simulink model "flightControlSystem"  (R2026b)
settings: Solver=ode3  StopTime=TFinal
PreLoadFcn:
  | InitVars;
  | definePX4ParamsBus;
undefined symbols (not defined in the file): control_power, DiscIntNeverNeededParam, init, MC_PITCHRATE_MAX, MC_ROLLRATE_MAX, MC_YAWRATE_MAX, PX4_Params_Default, SampleTime, timestamp
libraries: px4Utilslib x52, px4uORBlib x10, vrlib x8, aerolibutil x8, simulink x5, sharedutil x3, matrix_library x2, raspberrypiutilitieslib x2, px4Peripheralslib x2, sharedtransform x1, px4Sensorslib x1
(part 3 of 4)

== system flightControlSystem/MultiCopter Controller/Position & Altitude controller/Position controller/thrustToAttitude ==
  note: - Converts thrust vector to desired attitude (roll, pitch, yaw)
      | - Attitude setpoint is calculated so that the thrust vector aligns with desired acceleration
      | - Yaw setpoint (heading) is directly commanded
  thrust_setpoint_NED_3x1 : Inport
  yaw_setpoint_rad : Inport  Port=2
  Abs : Abs  SaturateOnIntegerOverflow=off
  Assignment : Assignment  DiagnosticForDimensions=Warning  IndexOptions=Index vector (dialog)  Indices=[3]  OutputSizes=1  RuntimeRangeChecks=off
  Assignment1 : Assignment  DiagnosticForDimensions=Warning  IndexOptions=Index vector (dialog)  Indices=3  OutputSizes=1  RuntimeRangeChecks=off
  Compare_Norm : RelationalOperator  Operator=<  OutDataTypeStr=boolean  RndMeth=Simplest  InputSameDT=off
  Constant : Constant  Value=eps  SampleTime=-1
  Constant1 : Constant  SampleTime=-1
  Constant2 : Constant  Value=0  SampleTime=-1
  Constant3 : Constant  Value=0.0  SampleTime=-1
  Constant4 : Constant  Value=1e-6  OutDataTypeStr=single  SampleTime=-1
  Constant5 : Constant  Value=single([0;0;1])  OutDataTypeStr=single  SampleTime=-1
  Cos_YawHeading : Trigonometry  Operator=cos
  Cross_BodyX_eq_Y_cross_Z : matrix_library/Cross Product
  Cross_BodyY_eq_Z_cross_Xdes : matrix_library/Cross Product
  Dot_CheckParallel : DotProduct  OutDataTypeStr=Inherit: Inherit via internal rule
  Gain : Gain  Gain=-1
  Gain1 : Gain  Gain=-1
  Mux_HeadingVector_cosYaw_sinYaw_0 : Mux  Inputs=3
  Negate_ThrustBodyFrame : Gain  Gain=-1
  Negate_ThrustForBodyZ : Gain  Gain=-1
  Normalize_BodyY : vrlib/Utilities/Normalize Vector  maxzero=0
  Normalize_BodyZ : vrlib/Utilities/Normalize Vector  maxzero=0
  Relational Operator : RelationalOperator  Operator=<  OutDataTypeStr=boolean  RndMeth=Simplest  InputSameDT=off
  Relational Operator1 : RelationalOperator  Operator=<  OutDataTypeStr=boolean  RndMeth=Simplest  InputSameDT=off
  RotMat_To_Euler_RPY : MATLAB Function  TreatAsAtomicUnit=on
  Selector : Selector  InputPortWidth=3  IndexOptions=Index vector (dialog)  Indices=3  OutputSizes=1  RuntimeRangeChecks=off
  Selector1 : Selector  InputPortWidth=3  IndexOptions=Index vector (dialog)  Indices=3  OutputSizes=1  RuntimeRangeChecks=off
  Sin_YawHeading : Trigonometry
  Switch_Singularity_BodyY : Switch  Criteria=u2 > Threshold  SaturateOnIntegerOverflow=off  InputSameDT=off
  Switch_Singularity_BodyZ : Switch  Criteria=u2 > Threshold  SaturateOnIntegerOverflow=off  InputSameDT=off
  Switch_Singularity_HeadingParallel : Switch  Criteria=u2 > Threshold  SaturateOnIntegerOverflow=off  InputSameDT=off
  ThrustMagnitude_Norm : MATLAB Function  TreatAsAtomicUnit=on
  attitude_euler_rpy_rad : Outport
  thrust_magnitude_normalized : Outport  Port=2
  thrust_body_frame_for_decoupling : Outport  Port=3
  wires:
  Switch_Singularity_HeadingParallel/1 -> Normalize_BodyY/1
  Gain/1 -> Switch_Singularity_BodyY/1
  Gain1/1 -> Assignment1/2
  Negate_ThrustBodyFrame/1 -> Mux_HeadingVector_cosYaw_sinYaw_0/1
  thrust_setpoint_NED_3x1/1 -> Assignment1/1, ThrustMagnitude_Norm/1(u), Negate_ThrustForBodyZ/1
  Constant/1 -> Compare_Norm/2
  Constant1/1 -> Assignment/2
  Selector1/1 -> thrust_body_frame_for_decoupling/1
  Sin_YawHeading/1 -> Negate_ThrustBodyFrame/1
  ThrustMagnitude_Norm/1(y) -> Gain1/1
  Dot_CheckParallel/1 -> Compare_Norm/1
  yaw_setpoint_rad/1 -> Cos_YawHeading/1, Sin_YawHeading/1
  Negate_ThrustForBodyZ/1 -> Dot_CheckParallel/2, Switch_Singularity_BodyZ/3, Assignment/1, Dot_CheckParallel/1
  Assignment/1 -> Switch_Singularity_BodyZ/1
  Assignment1/1 -> Selector1/1, thrust_magnitude_normalized/1
  Cos_YawHeading/1 -> Mux_HeadingVector_cosYaw_sinYaw_0/2
  Compare_Norm/1 -> Switch_Singularity_BodyZ/2
  Constant3/1 -> Relational Operator/2
  Constant2/1 -> Mux_HeadingVector_cosYaw_sinYaw_0/3
  Switch_Singularity_BodyZ/1 -> Normalize_BodyZ/1
  Mux_HeadingVector_cosYaw_sinYaw_0/1 -> Cross_BodyY_eq_Z_cross_Xdes/1
  Normalize_BodyZ/1 -> Cross_BodyX_eq_Y_cross_Z/1, RotMat_To_Euler_RPY/3(body_z), Selector/1, Cross_BodyY_eq_Z_cross_Xdes/2
  Selector/1 -> Abs/1, Relational Operator/1
  Cross_BodyY_eq_Z_cross_Xdes/1 -> Switch_Singularity_BodyY/3, Gain/1
  Abs/1 -> Relational Operator1/1
  Relational Operator1/1 -> Switch_Singularity_HeadingParallel/2
  Constant5/1 -> Switch_Singularity_HeadingParallel/1
  Constant4/1 -> Relational Operator1/2
  Relational Operator/1 -> Switch_Singularity_BodyY/2
  Switch_Singularity_BodyY/1 -> Switch_Singularity_HeadingParallel/3
  Normalize_BodyY/1 -> RotMat_To_Euler_RPY/1(body_x), Cross_BodyX_eq_Y_cross_Z/2
  Cross_BodyX_eq_Y_cross_Z/1 -> RotMat_To_Euler_RPY/2(body_y)
  RotMat_To_Euler_RPY/1(y) -> attitude_euler_rpy_rad/1

== system flightControlSystem/ParamUpdate/HW_ParamUpdate/ReadParams_OnUpdate/AttitudeCtrl_Params ==
  Cast_Mux_MC_ATT_P : DataTypeConversion  OutDataTypeStr=double  SaturateOnIntegerOverflow=off  RndMeth=Floor
  Cast_RP_MC_YAW_WEIGHT : DataTypeConversion  OutDataTypeStr=double  SaturateOnIntegerOverflow=off  RndMeth=Floor
  Mux_MC_ATT_P : Mux  Inputs=3
  RP_MC_ATT_P_1 : px4Utilslib/Read Parameter  ParameterName=MC_ROLL_P  DataType=FLOAT  SampleTime=-1
  RP_MC_ATT_P_2 : px4Utilslib/Read Parameter  ParameterName=MC_PITCH_P  DataType=FLOAT  SampleTime=-1
  RP_MC_ATT_P_3 : px4Utilslib/Read Parameter  ParameterName=MC_YAW_P  DataType=FLOAT  SampleTime=-1
  RP_MC_YAW_WEIGHT : px4Utilslib/Read Parameter  ParameterName=MC_YAW_WEIGHT  DataType=FLOAT  SampleTime=-1
  Term_Status{,1..3} (4 alike) : Terminator
  MC_ATT_P : Outport
  MC_YAW_WEIGHT : Outport  Port=2
  wires:
  RP_MC_ATT_P_3/2 -> Term_Status3/1
  RP_MC_ATT_P_2/2 -> Term_Status2/1
  RP_MC_ATT_P_1/2 -> Term_Status1/1
  RP_MC_YAW_WEIGHT/2 -> Term_Status/1
  RP_MC_ATT_P_3/1 -> Mux_MC_ATT_P/3
  Mux_MC_ATT_P/1 -> Cast_Mux_MC_ATT_P/1
  RP_MC_ATT_P_2/1 -> Mux_MC_ATT_P/2
  Cast_RP_MC_YAW_WEIGHT/1 -> MC_YAW_WEIGHT/1
  RP_MC_YAW_WEIGHT/1 -> Cast_RP_MC_YAW_WEIGHT/1
  Cast_Mux_MC_ATT_P/1 -> MC_ATT_P/1
  RP_MC_ATT_P_1/1 -> Mux_MC_ATT_P/1

== system flightControlSystem/ParamUpdate/HW_ParamUpdate/ReadParams_OnUpdate/Estimator_Params ==
  Cast_RP_MPC_VELD_LP : DataTypeConversion  OutDataTypeStr=double  SaturateOnIntegerOverflow=off  RndMeth=Floor
  EST_NF_BW_Const : Constant  Value=20  SampleTime=-1
  EST_NF_FRQ_Const : Constant  Value=30  SampleTime=-1
  RP_MPC_VELD_LP : px4Utilslib/Read Parameter  ParameterName=MPC_VELD_LP  DataType=FLOAT  SampleTime=-1
  Term_Status : Terminator
  MPC_VELD_LP : Outport
  EST_NF_FRQ : Outport  Port=2
  EST_NF_BW : Outport  Port=3
  wires:
  EST_NF_BW_Const/1 -> EST_NF_BW/1
  RP_MPC_VELD_LP/2 -> Term_Status/1
  Cast_RP_MPC_VELD_LP/1 -> MPC_VELD_LP/1
  RP_MPC_VELD_LP/1 -> Cast_RP_MPC_VELD_LP/1
  EST_NF_FRQ_Const/1 -> EST_NF_FRQ/1

== system flightControlSystem/ParamUpdate/HW_ParamUpdate/ReadParams_OnUpdate/LandingLogic_Params ==
  Cast_RP_MPC_LAND_ALT1 : DataTypeConversion  OutDataTypeStr=double  SaturateOnIntegerOverflow=off  RndMeth=Floor
  Cast_RP_MPC_LAND_ALT2 : DataTypeConversion  OutDataTypeStr=double  SaturateOnIntegerOverflow=off  RndMeth=Floor
  Cast_RP_MPC_LAND_ALT3 : DataTypeConversion  OutDataTypeStr=double  SaturateOnIntegerOverflow=off  RndMeth=Floor
  Cast_RP_MPC_LAND_CRWL : DataTypeConversion  OutDataTypeStr=double  SaturateOnIntegerOverflow=off  RndMeth=Floor
  Cast_RP_MPC_LAND_SPEED : DataTypeConversion  OutDataTypeStr=double  SaturateOnIntegerOverflow=off  RndMeth=Floor
  Cast_RP_MPC_Z_VEL_MAX_DN_LAND : DataTypeConversion  OutDataTypeStr=double  SaturateOnIntegerOverflow=off  RndMeth=Floor
  RP_MPC_LAND_ALT1 : px4Utilslib/Read Parameter  ParameterName=MPC_LAND_ALT1  DataType=FLOAT  SampleTime=-1
  RP_MPC_LAND_ALT2 : px4Utilslib/Read Parameter  ParameterName=MPC_LAND_ALT2  DataType=FLOAT  SampleTime=-1
  RP_MPC_LAND_ALT3 : px4Utilslib/Read Parameter  ParameterName=MPC_LAND_ALT3  DataType=FLOAT  SampleTime=-1
  RP_MPC_LAND_CRWL : px4Utilslib/Read Parameter  ParameterName=MPC_LAND_CRWL  DataType=FLOAT  SampleTime=-1
  RP_MPC_LAND_SPEED : px4Utilslib/Read Parameter  ParameterName=MPC_LAND_SPEED  DataType=FLOAT  SampleTime=-1
  RP_MPC_Z_VEL_MAX_DN_LAND : px4Utilslib/Read Parameter  ParameterName=MPC_Z_VEL_MAX_DN  DataType=FLOAT  SampleTime=-1
  Term_Out{2..3,5..6,8..9} (6 alike) : Terminator
  Term_Status{,1..5} (6 alike) : Terminator
  MPC_LAND_ALT1 : Outport
  MPC_LAND_ALT2 : Outport  Port=2
  MPC_LAND_ALT3 : Outport  Port=3
  MPC_LAND_SPEED : Outport  Port=4
  MPC_LAND_CRWL : Outport  Port=5
  MPC_Z_VEL_MAX_DN_LAND : Outport  Port=6
  wires:
  RP_MPC_Z_VEL_MAX_DN_LAND/2 -> Term_Status5/1
  RP_MPC_LAND_CRWL/2 -> Term_Status4/1
  RP_MPC_LAND_SPEED/2 -> Term_Status3/1
  Cast_RP_MPC_Z_VEL_MAX_DN_LAND/1 -> MPC_Z_VEL_MAX_DN_LAND/1, Term_Out9/1
  Cast_RP_MPC_LAND_CRWL/1 -> MPC_LAND_CRWL/1, Term_Out8/1
  RP_MPC_LAND_ALT3/2 -> Term_Status2/1
  Cast_RP_MPC_LAND_SPEED/1 -> MPC_LAND_SPEED/1, Term_Out6/1
  Cast_RP_MPC_LAND_ALT3/1 -> MPC_LAND_ALT3/1, Term_Out5/1
  RP_MPC_LAND_ALT2/2 -> Term_Status1/1
  Cast_RP_MPC_LAND_ALT2/1 -> MPC_LAND_ALT2/1, Term_Out3/1
  Cast_RP_MPC_LAND_ALT1/1 -> MPC_LAND_ALT1/1, Term_Out2/1
  RP_MPC_LAND_ALT1/2 -> Term_Status/1
  RP_MPC_LAND_CRWL/1 -> Cast_RP_MPC_LAND_CRWL/1
  RP_MPC_LAND_SPEED/1 -> Cast_RP_MPC_LAND_SPEED/1
  RP_MPC_LAND_ALT2/1 -> Cast_RP_MPC_LAND_ALT2/1
  RP_MPC_LAND_ALT3/1 -> Cast_RP_MPC_LAND_ALT3/1
  RP_MPC_Z_VEL_MAX_DN_LAND/1 -> Cast_RP_MPC_Z_VEL_MAX_DN_LAND/1
  RP_MPC_LAND_ALT1/1 -> Cast_RP_MPC_LAND_ALT1/1

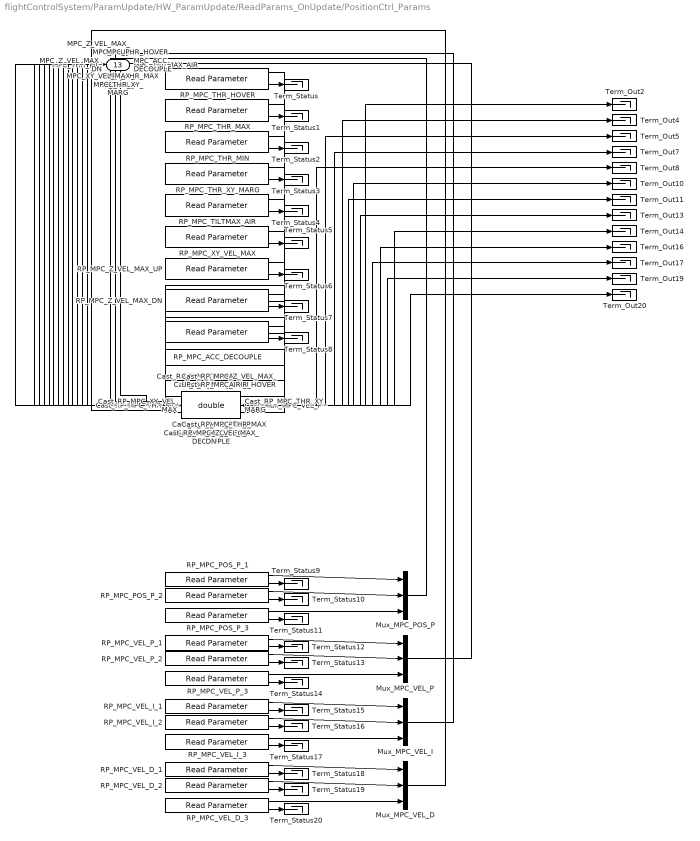
== system flightControlSystem/ParamUpdate/HW_ParamUpdate/ReadParams_OnUpdate/PositionCtrl_Params ==
  Cast_Mux_MPC_POS_P : DataTypeConversion  OutDataTypeStr=double  SaturateOnIntegerOverflow=off  RndMeth=Floor
  Cast_Mux_MPC_VEL_D : DataTypeConversion  OutDataTypeStr=double  SaturateOnIntegerOverflow=off  RndMeth=Floor
  Cast_Mux_MPC_VEL_I : DataTypeConversion  OutDataTypeStr=double  SaturateOnIntegerOverflow=off  RndMeth=Floor
  Cast_Mux_MPC_VEL_P : DataTypeConversion  OutDataTypeStr=double  SaturateOnIntegerOverflow=off  RndMeth=Floor
  Cast_RP_MPC_ACC_DECOUPLE : DataTypeConversion  OutDataTypeStr=double  SaturateOnIntegerOverflow=off  RndMeth=Floor
  Cast_RP_MPC_THR_HOVER : DataTypeConversion  OutDataTypeStr=double  SaturateOnIntegerOverflow=off  RndMeth=Floor
  Cast_RP_MPC_THR_MAX : DataTypeConversion  OutDataTypeStr=double  SaturateOnIntegerOverflow=off  RndMeth=Floor
  Cast_RP_MPC_THR_MIN : DataTypeConversion  OutDataTypeStr=double  SaturateOnIntegerOverflow=off  RndMeth=Floor
  Cast_RP_MPC_THR_XY_MARG : DataTypeConversion  OutDataTypeStr=double  SaturateOnIntegerOverflow=off  RndMeth=Floor
  Cast_RP_MPC_TILTMAX_AIR : DataTypeConversion  OutDataTypeStr=double  SaturateOnIntegerOverflow=off  RndMeth=Floor
  Cast_RP_MPC_XY_VEL_MAX : DataTypeConversion  OutDataTypeStr=double  SaturateOnIntegerOverflow=off  RndMeth=Floor
  Cast_RP_MPC_Z_VEL_MAX_DN : DataTypeConversion  OutDataTypeStr=double  SaturateOnIntegerOverflow=off  RndMeth=Floor
  Cast_RP_MPC_Z_VEL_MAX_UP : DataTypeConversion  OutDataTypeStr=double  SaturateOnIntegerOverflow=off  RndMeth=Floor
  Mux_MPC_POS_P : Mux  Inputs=3
  Mux_MPC_VEL_D : Mux  Inputs=3
  Mux_MPC_VEL_I : Mux  Inputs=3
  Mux_MPC_VEL_P : Mux  Inputs=3
  RP_MPC_ACC_DECOUPLE : px4Utilslib/Read Parameter  ParameterName=MPC_ACC_DECOUPLE  DataType=INT32  SampleTime=-1
  RP_MPC_POS_P_1 : px4Utilslib/Read Parameter  ParameterName=MPC_XY_P  DataType=FLOAT  SampleTime=-1
  RP_MPC_POS_P_2 : px4Utilslib/Read Parameter  ParameterName=MPC_XY_P  DataType=FLOAT  SampleTime=-1
  RP_MPC_POS_P_3 : px4Utilslib/Read Parameter  ParameterName=MPC_Z_P  DataType=FLOAT  SampleTime=-1
  RP_MPC_THR_HOVER : px4Utilslib/Read Parameter  ParameterName=MPC_THR_HOVER  DataType=FLOAT  SampleTime=-1
  RP_MPC_THR_MAX : px4Utilslib/Read Parameter  ParameterName=MPC_THR_MAX  DataType=FLOAT  SampleTime=-1
  RP_MPC_THR_MIN : px4Utilslib/Read Parameter  ParameterName=MPC_THR_MIN  DataType=FLOAT  SampleTime=-1
  RP_MPC_THR_XY_MARG : px4Utilslib/Read Parameter  ParameterName=MPC_THR_XY_MARG  DataType=FLOAT  SampleTime=-1
  RP_MPC_TILTMAX_AIR : px4Utilslib/Read Parameter  ParameterName=MPC_TILTMAX_AIR  DataType=FLOAT  SampleTime=-1
  RP_MPC_VEL_D_1 : px4Utilslib/Read Parameter  ParameterName=MPC_XY_VEL_D_ACC  DataType=FLOAT  SampleTime=-1
  RP_MPC_VEL_D_2 : px4Utilslib/Read Parameter  ParameterName=MPC_XY_VEL_D_ACC  DataType=FLOAT  SampleTime=-1
  RP_MPC_VEL_D_3 : px4Utilslib/Read Parameter  ParameterName=MPC_Z_VEL_D_ACC  DataType=FLOAT  SampleTime=-1
  RP_MPC_VEL_I_1 : px4Utilslib/Read Parameter  ParameterName=MPC_XY_VEL_I_ACC  DataType=FLOAT  SampleTime=-1
  RP_MPC_VEL_I_2 : px4Utilslib/Read Parameter  ParameterName=MPC_XY_VEL_I_ACC  DataType=FLOAT  SampleTime=-1
  RP_MPC_VEL_I_3 : px4Utilslib/Read Parameter  ParameterName=MPC_Z_VEL_I_ACC  DataType=FLOAT  SampleTime=-1
  RP_MPC_VEL_P_1 : px4Utilslib/Read Parameter  ParameterName=MPC_XY_VEL_P_ACC  DataType=FLOAT  SampleTime=-1
  RP_MPC_VEL_P_2 : px4Utilslib/Read Parameter  ParameterName=MPC_XY_VEL_P_ACC  DataType=FLOAT  SampleTime=-1
  RP_MPC_VEL_P_3 : px4Utilslib/Read Parameter  ParameterName=MPC_Z_VEL_P_ACC  DataType=FLOAT  SampleTime=-1
  RP_MPC_XY_VEL_MAX : px4Utilslib/Read Parameter  ParameterName=MPC_XY_VEL_MAX  DataType=FLOAT  SampleTime=-1
  RP_MPC_Z_VEL_MAX_DN : px4Utilslib/Read Parameter  ParameterName=MPC_Z_VEL_MAX_DN  DataType=FLOAT  SampleTime=-1
  RP_MPC_Z_VEL_MAX_UP : px4Utilslib/Read Parameter  ParameterName=MPC_Z_VEL_MAX_UP  DataType=FLOAT  SampleTime=-1
  Term_Out{2,4..5,7..8,10..11,13..14,16..17,19..20} (13 alike) : Terminator
  Term_Status{,1..20} (21 alike) : Terminator
  MPC_POS_P : Outport
  MPC_VEL_P : Outport  Port=2
  MPC_VEL_I : Outport  Port=3
  MPC_VEL_D : Outport  Port=4
  MPC_THR_HOVER : Outport  Port=5
  MPC_THR_MAX : Outport  Port=6
  MPC_THR_MIN : Outport  Port=7
  MPC_THR_XY_MARG : Outport  Port=8
  MPC_TILTMAX_AIR : Outport  Port=9
  MPC_XY_VEL_MAX : Outport  Port=10
  MPC_Z_VEL_MAX_UP : Outport  Port=11
  MPC_Z_VEL_MAX_DN : Outport  Port=12
  MPC_ACC_DECOUPLE : Outport  Port=13
  wires:
  RP_MPC_VEL_D_3/2 -> Term_Status20/1
  RP_MPC_VEL_D_2/2 -> Term_Status19/1
  RP_MPC_VEL_D_1/2 -> Term_Status18/1
  RP_MPC_VEL_I_3/2 -> Term_Status17/1
  RP_MPC_VEL_I_2/2 -> Term_Status16/1
  RP_MPC_VEL_I_1/2 -> Term_Status15/1
  RP_MPC_VEL_P_3/2 -> Term_Status14/1
  RP_MPC_VEL_P_2/2 -> Term_Status13/1
  RP_MPC_VEL_P_1/2 -> Term_Status12/1
  RP_MPC_POS_P_3/2 -> Term_Status11/1
  RP_MPC_POS_P_2/2 -> Term_Status10/1
  RP_MPC_POS_P_1/2 -> Term_Status9/1
  RP_MPC_ACC_DECOUPLE/2 -> Term_Status8/1
  RP_MPC_Z_VEL_MAX_DN/2 -> Term_Status7/1
  Cast_RP_MPC_ACC_DECOUPLE/1 -> MPC_ACC_DECOUPLE/1, Term_Out20/1
  Cast_RP_MPC_Z_VEL_MAX_DN/1 -> MPC_Z_VEL_MAX_DN/1, Term_Out19/1
  RP_MPC_Z_VEL_MAX_UP/2 -> Term_Status6/1
  Cast_RP_MPC_Z_VEL_MAX_UP/1 -> MPC_Z_VEL_MAX_UP/1, Term_Out17/1
  Cast_RP_MPC_XY_VEL_MAX/1 -> MPC_XY_VEL_MAX/1, Term_Out16/1
  RP_MPC_XY_VEL_MAX/2 -> Term_Status5/1
  Cast_RP_MPC_TILTMAX_AIR/1 -> MPC_TILTMAX_AIR/1, Term_Out14/1
  Cast_RP_MPC_THR_XY_MARG/1 -> MPC_THR_XY_MARG/1, Term_Out13/1
  RP_MPC_TILTMAX_AIR/2 -> Term_Status4/1
  Cast_RP_MPC_THR_MIN/1 -> MPC_THR_MIN/1, Term_Out11/1
  Cast_RP_MPC_THR_MAX/1 -> MPC_THR_MAX/1, Term_Out10/1
  RP_MPC_THR_XY_MARG/2 -> Term_Status3/1
  Cast_RP_MPC_THR_HOVER/1 -> MPC_THR_HOVER/1, Term_Out8/1
  Cast_Mux_MPC_VEL_D/1 -> MPC_VEL_D/1, Term_Out7/1
  RP_MPC_THR_MIN/2 -> Term_Status2/1
  Cast_Mux_MPC_VEL_I/1 -> MPC_VEL_I/1, Term_Out5/1
  Cast_Mux_MPC_VEL_P/1 -> MPC_VEL_P/1, Term_Out4/1
  RP_MPC_THR_MAX/2 -> Term_Status1/1
  Cast_Mux_MPC_POS_P/1 -> MPC_POS_P/1, Term_Out2/1
  RP_MPC_THR_HOVER/2 -> Term_Status/1
  RP_MPC_VEL_D_2/1 -> Mux_MPC_VEL_D/2
  RP_MPC_VEL_P_3/1 -> Mux_MPC_VEL_P/3
  RP_MPC_VEL_I_2/1 -> Mux_MPC_VEL_I/2
  Mux_MPC_VEL_P/1 -> Cast_Mux_MPC_VEL_P/1
  Mux_MPC_POS_P/1 -> Cast_Mux_MPC_POS_P/1
  RP_MPC_POS_P_2/1 -> Mux_MPC_POS_P/2
  Mux_MPC_VEL_I/1 -> Cast_Mux_MPC_VEL_I/1
  RP_MPC_POS_P_1/1 -> Mux_MPC_POS_P/1
  RP_MPC_VEL_I_1/1 -> Mux_MPC_VEL_I/1
  RP_MPC_Z_VEL_MAX_DN/1 -> Cast_RP_MPC_Z_VEL_MAX_DN/1
  RP_MPC_THR_XY_MARG/1 -> Cast_RP_MPC_THR_XY_MARG/1
  RP_MPC_POS_P_3/1 -> Mux_MPC_POS_P/3
  Mux_MPC_VEL_D/1 -> Cast_Mux_MPC_VEL_D/1
  RP_MPC_VEL_D_1/1 -> Mux_MPC_VEL_D/1
  RP_MPC_THR_MIN/1 -> Cast_RP_MPC_THR_MIN/1
  RP_MPC_THR_MAX/1 -> Cast_RP_MPC_THR_MAX/1
  RP_MPC_Z_VEL_MAX_UP/1 -> Cast_RP_MPC_Z_VEL_MAX_UP/1
  RP_MPC_VEL_I_3/1 -> Mux_MPC_VEL_I/3
  RP_MPC_VEL_D_3/1 -> Mux_MPC_VEL_D/3
  RP_MPC_VEL_P_1/1 -> Mux_MPC_VEL_P/1
  RP_MPC_ACC_DECOUPLE/1 -> Cast_RP_MPC_ACC_DECOUPLE/1
  RP_MPC_THR_HOVER/1 -> Cast_RP_MPC_THR_HOVER/1
  RP_MPC_XY_VEL_MAX/1 -> Cast_RP_MPC_XY_VEL_MAX/1
  RP_MPC_VEL_P_2/1 -> Mux_MPC_VEL_P/2
  RP_MPC_TILTMAX_AIR/1 -> Cast_RP_MPC_TILTMAX_AIR/1

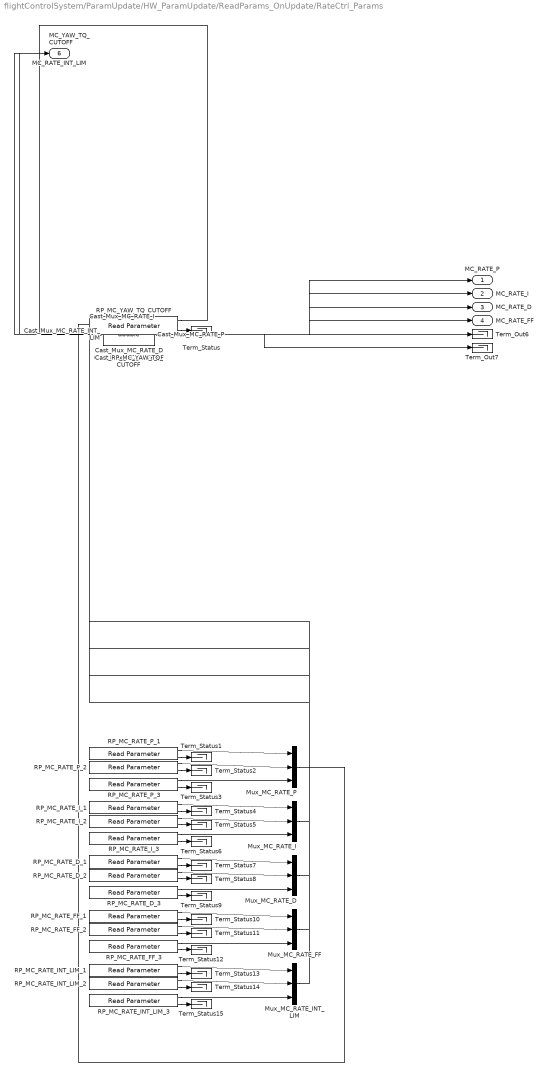
== system flightControlSystem/ParamUpdate/HW_ParamUpdate/ReadParams_OnUpdate/RateCtrl_Params ==
  Cast_Mux_MC_RATE_D : DataTypeConversion  OutDataTypeStr=double  SaturateOnIntegerOverflow=off  RndMeth=Floor
  Cast_Mux_MC_RATE_FF : DataTypeConversion  OutDataTypeStr=double  SaturateOnIntegerOverflow=off  RndMeth=Floor
  Cast_Mux_MC_RATE_I : DataTypeConversion  OutDataTypeStr=double  SaturateOnIntegerOverflow=off  RndMeth=Floor
  Cast_Mux_MC_RATE_INT_LIM : DataTypeConversion  OutDataTypeStr=double  SaturateOnIntegerOverflow=off  RndMeth=Floor
  Cast_Mux_MC_RATE_P : DataTypeConversion  OutDataTypeStr=double  SaturateOnIntegerOverflow=off  RndMeth=Floor
  Cast_RP_MC_YAW_TQ_CUTOFF : DataTypeConversion  OutDataTypeStr=double  SaturateOnIntegerOverflow=off  RndMeth=Floor
  Mux_MC_RATE_D : Mux  Inputs=3
  Mux_MC_RATE_FF : Mux  Inputs=3
  Mux_MC_RATE_I : Mux  Inputs=3
  Mux_MC_RATE_INT_LIM : Mux  Inputs=3
  Mux_MC_RATE_P : Mux  Inputs=3
  RP_MC_RATE_D_1 : px4Utilslib/Read Parameter  ParameterName=MC_ROLLRATE_D  DataType=FLOAT  SampleTime=-1
  RP_MC_RATE_D_2 : px4Utilslib/Read Parameter  ParameterName=MC_PITCHRATE_D  DataType=FLOAT  SampleTime=-1
  RP_MC_RATE_D_3 : px4Utilslib/Read Parameter  ParameterName=MC_YAWRATE_D  DataType=FLOAT  SampleTime=-1
  RP_MC_RATE_FF_1 : px4Utilslib/Read Parameter  ParameterName=MC_ROLLRATE_FF  DataType=FLOAT  SampleTime=-1
  RP_MC_RATE_FF_2 : px4Utilslib/Read Parameter  ParameterName=MC_PITCHRATE_FF  DataType=FLOAT  SampleTime=-1
  RP_MC_RATE_FF_3 : px4Utilslib/Read Parameter  ParameterName=MC_YAWRATE_FF  DataType=FLOAT  SampleTime=-1
  RP_MC_RATE_INT_LIM_1 : px4Utilslib/Read Parameter  ParameterName=MC_RR_INT_LIM  DataType=FLOAT  SampleTime=-1
  RP_MC_RATE_INT_LIM_2 : px4Utilslib/Read Parameter  ParameterName=MC_PR_INT_LIM  DataType=FLOAT  SampleTime=-1
  RP_MC_RATE_INT_LIM_3 : px4Utilslib/Read Parameter  ParameterName=MC_YR_INT_LIM  DataType=FLOAT  SampleTime=-1
  RP_MC_RATE_I_1 : px4Utilslib/Read Parameter  ParameterName=MC_ROLLRATE_I  DataType=FLOAT  SampleTime=-1
  RP_MC_RATE_I_2 : px4Utilslib/Read Parameter  ParameterName=MC_PITCHRATE_I  DataType=FLOAT  SampleTime=-1
  RP_MC_RATE_I_3 : px4Utilslib/Read Parameter  ParameterName=MC_YAWRATE_I  DataType=FLOAT  SampleTime=-1
  RP_MC_RATE_P_1 : px4Utilslib/Read Parameter  ParameterName=MC_ROLLRATE_P  DataType=FLOAT  SampleTime=-1
  RP_MC_RATE_P_2 : px4Utilslib/Read Parameter  ParameterName=MC_PITCHRATE_P  DataType=FLOAT  SampleTime=-1
  RP_MC_RATE_P_3 : px4Utilslib/Read Parameter  ParameterName=MC_YAWRATE_P  DataType=FLOAT  SampleTime=-1
  RP_MC_YAW_TQ_CUTOFF : px4Utilslib/Read Parameter  ParameterName=MC_YAW_TQ_CUTOFF  DataType=FLOAT  SampleTime=-1
  Term_Out6 : Terminator
  Term_Out7 : Terminator
  Term_Status{,1..15} (16 alike) : Terminator
  MC_RATE_P : Outport
  MC_RATE_I : Outport  Port=2
  MC_RATE_D : Outport  Port=3
  MC_RATE_FF : Outport  Port=4
  MC_RATE_INT_LIM : Outport  Port=5
  MC_YAW_TQ_CUTOFF : Outport  Port=6
  wires:
  RP_MC_RATE_INT_LIM_3/2 -> Term_Status15/1
  RP_MC_RATE_INT_LIM_2/2 -> Term_Status14/1
  RP_MC_RATE_INT_LIM_1/2 -> Term_Status13/1
  RP_MC_RATE_FF_3/2 -> Term_Status12/1
  RP_MC_RATE_FF_2/2 -> Term_Status11/1
  RP_MC_RATE_FF_1/2 -> Term_Status10/1
  RP_MC_RATE_D_3/2 -> Term_Status9/1
  RP_MC_RATE_D_2/2 -> Term_Status8/1
  RP_MC_RATE_D_1/2 -> Term_Status7/1
  RP_MC_RATE_I_3/2 -> Term_Status6/1
  RP_MC_RATE_I_2/2 -> Term_Status5/1
  RP_MC_RATE_I_1/2 -> Term_Status4/1
  RP_MC_RATE_P_3/2 -> Term_Status3/1
  RP_MC_RATE_P_2/2 -> Term_Status2/1
  RP_MC_RATE_P_1/2 -> Term_Status1/1
  Cast_RP_MC_YAW_TQ_CUTOFF/1 -> MC_YAW_TQ_CUTOFF/1, Term_Out7/1
  Cast_Mux_MC_RATE_INT_LIM/1 -> MC_RATE_INT_LIM/1, Term_Out6/1
  RP_MC_YAW_TQ_CUTOFF/2 -> Term_Status/1
  Cast_Mux_MC_RATE_D/1 -> MC_RATE_D/1
  Cast_Mux_MC_RATE_I/1 -> MC_RATE_I/1
  Cast_Mux_MC_RATE_P/1 -> MC_RATE_P/1
  Mux_MC_RATE_INT_LIM/1 -> Cast_Mux_MC_RATE_INT_LIM/1
  RP_MC_RATE_INT_LIM_1/1 -> Mux_MC_RATE_INT_LIM/1
  RP_MC_RATE_FF_3/1 -> Mux_MC_RATE_FF/3
  Mux_MC_RATE_FF/1 -> Cast_Mux_MC_RATE_FF/1
  RP_MC_RATE_FF_2/1 -> Mux_MC_RATE_FF/2
  RP_MC_RATE_INT_LIM_2/1 -> Mux_MC_RATE_INT_LIM/2
  RP_MC_RATE_I_3/1 -> Mux_MC_RATE_I/3
  Mux_MC_RATE_I/1 -> Cast_Mux_MC_RATE_I/1
  RP_MC_RATE_I_1/1 -> Mux_MC_RATE_I/1
  RP_MC_RATE_D_2/1 -> Mux_MC_RATE_D/2
  Mux_MC_RATE_D/1 -> Cast_Mux_MC_RATE_D/1
  RP_MC_RATE_INT_LIM_3/1 -> Mux_MC_RATE_INT_LIM/3
  RP_MC_RATE_P_3/1 -> Mux_MC_RATE_P/3
  RP_MC_RATE_I_2/1 -> Mux_MC_RATE_I/2
  RP_MC_RATE_D_3/1 -> Mux_MC_RATE_D/3
  Mux_MC_RATE_P/1 -> Cast_Mux_MC_RATE_P/1
  RP_MC_RATE_P_2/1 -> Mux_MC_RATE_P/2
  RP_MC_RATE_D_1/1 -> Mux_MC_RATE_D/1
  RP_MC_YAW_TQ_CUTOFF/1 -> Cast_RP_MC_YAW_TQ_CUTOFF/1
  Cast_Mux_MC_RATE_FF/1 -> MC_RATE_FF/1
  RP_MC_RATE_P_1/1 -> Mux_MC_RATE_P/1
  RP_MC_RATE_FF_1/1 -> Mux_MC_RATE_FF/1

== system flightControlSystem/SetpointManager/Set target Position/Setpoints from Perception Module/Enabled Subsystem ==
  CurrentPosition : Inport
  Enable : EnablePort
  Cast To Single : DataTypeConversion  OutDataTypeStr=single  SaturateOnIntegerOverflow=off  RndMeth=Floor
  Constant : Constant  Value=221  OutDataTypeStr=single  SampleTime=-1
  Demux : Demux
  Protocol Encoder : raspberrypiutilitieslib/Protocol Encoder  Header=[123]  FieldTable={ 'Field1', '1', 'single', 'Little endian'; 'Field2', '1', 'single', 'Little endian'; 'Field3', '1', 'single', 'Little endian'; 'Field4', '1', 'single', 'Little endian'; 'Field5', '1', 'single', 'Little endian' }  IsChecksumRequired=off  ChecksumAlgorithm=XOR of bytes  ChecksumSize=[]  TerminatorOption=<none>  CustomTerminatorVal=[]
  Selector : Selector  InputPortWidth=5  IndexOptions=Index vector (dialog)  Indices=[1:4]  OutputSizes=1  RuntimeRangeChecks=off
  Serial Transmit : px4Peripheralslib/Serial Transmit  SCIModule=/dev/ttyACM0
  wires:
  CurrentPosition/1 -> Selector/1
  Cast To Single/1 -> Demux/1
  Constant/1 -> Protocol Encoder/5
  Selector/1 -> Cast To Single/1
  Demux/1 -> Protocol Encoder/1
  Demux/2 -> Protocol Encoder/2
  Demux/3 -> Protocol Encoder/3
  Demux/4 -> Protocol Encoder/4
  Protocol Encoder/1 -> Serial Transmit/1

== system flightControlSystem/MultiCopter Controller/Angular Rate Control/RatePID_Core/ActuatorSaturation_Detector/If Action Subsystem1 ==
  Action Port : ActionPort  ActionPortLabel=else
  Constant1 : Constant  Value=[0, 0, 0]  OutDataTypeStr=boolean  SampleTime=-1
  Constant2 : Constant  Value=[0, 0, 0]  OutDataTypeStr=boolean  SampleTime=-1
  saturation_positive : Outport
  saturation_negative : Outport  Port=2
  wires:
  Constant2/1 -> saturation_positive/1
  Constant1/1 -> saturation_negative/1

== system flightControlSystem/MultiCopter Controller/Angular Rate Control/RatePID_Core/ActuatorSaturation_Detector/Subsystem1 ==
  unallocated_torque : Inport
  Action Port : ActionPort  ActionPortLabel=if(u1 ~= 0)
  Constant1 : Constant  Value=eps  SampleTime=-1
  Constant3 : Constant  Value=-eps  SampleTime=-1
  Relational Operator1 : RelationalOperator  Operator=>  OutDataTypeStr=boolean  RndMeth=Simplest  InputSameDT=off
  Relational Operator2 : RelationalOperator  Operator=<  OutDataTypeStr=boolean  RndMeth=Simplest  InputSameDT=off
  saturation_positive : Outport
  saturation_negative : Outport  Port=2
  wires:
  Relational Operator2/1 -> saturation_negative/1
  Constant1/1 -> Relational Operator1/2
  unallocated_torque/1 -> Relational Operator2/1, Relational Operator1/1
  Constant3/1 -> Relational Operator2/2
  Relational Operator1/1 -> saturation_positive/1

== system flightControlSystem/MultiCopter Controller/Angular Rate Control/RatePID_Core/rate_integral/AntiWindup_IntegralUpdate ==
  is_saturated_positive_3x1 : Inport
  is_saturated_negative_3x1 : Inport  Port=2
  gain_I_per_axis : Inport  Port=3
  integral_limit_symmetric : Inport  Port=4
  rate_error_rads : Inport  Port=5
  integral_state_prev : Inport  Port=6
  dt_s : Inport  Port=7
  Action Port : ActionPort  ActionPortLabel=if(u1 ~=0)
  Update_Integral : Subsystem  TreatAsAtomicUnit=on
  integral_state_new : Outport
  wires:
  rate_error_rads/1 -> Update_Integral/5(rate_error_scalar_rads)
  is_saturated_positive_3x1/1 -> Update_Integral/1(saturated_positive_bool)
  integral_state_prev/1 -> Update_Integral/6(integral_prev_scalar)
  is_saturated_negative_3x1/1 -> Update_Integral/2(saturated_negative_bool)
  gain_I_per_axis/1 -> Update_Integral/3(I_gain_scalar)
  dt_s/1 -> Update_Integral/7(dt_s)
  integral_limit_symmetric/1 -> Update_Integral/4(integral_limit)
  Update_Integral/1(integral_updated_scalar) -> integral_state_new/1

== system flightControlSystem/MultiCopter Controller/Angular Rate Control/RatePID_Core/rate_integral/IfLanded_ResetIntegral_PassZero ==
  rate_int_in : Inport
  Action Port : ActionPort  ActionPortLabel=else
  Out1 : Outport
  wires:
  rate_int_in/1 -> Out1/1

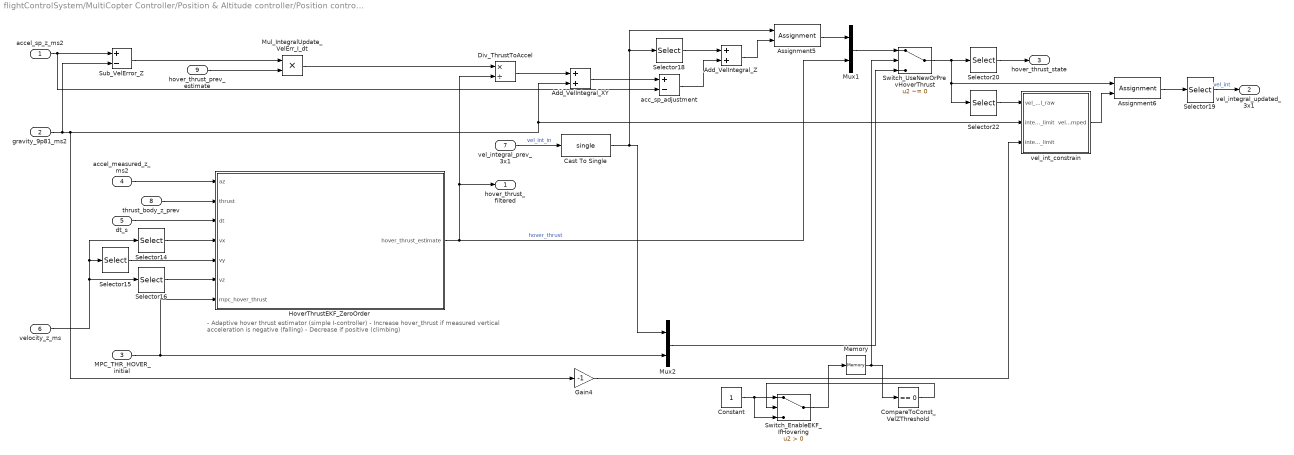
== system flightControlSystem/MultiCopter Controller/Position & Altitude controller/Position controller/PositionVelocityControl/Hover_Thrust ==
  note: - Adaptive hover thrust estimator (simple I-controller)
      | - Increase hover_thrust if measured vertical acceleration is negative (falling)
      | - Decrease if positive (climbing)
  accel_sp_z_ms2 : Inport
  gravity_9p81_ms2 : Inport  Port=2
  MPC_THR_HOVER_initial : Inport  Port=3
  accel_measured_z_ms2 : Inport  Port=4
  dt_s : Inport  Port=5
  velocity_z_ms : Inport  Port=6
  vel_integral_prev_3x1 : Inport  Port=7
  thrust_body_z_prev : Inport  Port=8
  hover_thrust_prev_estimate : Inport  Port=9
  Add_VelIntegral_XY : Sum
  Add_VelIntegral_Z : Sum
  Assignment5 : Assignment  DiagnosticForDimensions=Warning  IndexOptions=Index vector (dialog)  Indices=3  OutputSizes=1  RuntimeRangeChecks=off
  Assignment6 : Assignment  DiagnosticForDimensions=Warning  IndexOptions=Index vector (dialog)  Indices=3  OutputSizes=1  RuntimeRangeChecks=off
  Cast To Single : DataTypeConversion  OutDataTypeStr=single  SaturateOnIntegerOverflow=off  RndMeth=Floor
  CompareToConst_VelZThreshold : simulink/Logic and Bit Operations/Compare To Constant  relop===  const=0  OutDataTypeStr=boolean
  Constant : Constant  SampleTime=-1
  Div_ThrustToAccel : Product  Inputs=*/
  Gain4 : Gain  Gain=-1
  HoverThrustEKF_ZeroOrder : MATLAB Function  TreatAsAtomicUnit=on
  Memory : Memory  InheritSampleTime=on
  Mul_IntegralUpdate_VelErr_I_dt : Product
  Mux1 : Mux  Inputs=2
  Mux2 : Mux  Inputs=2
  Selector14 : Selector  InputPortWidth=3  IndexOptions=Index vector (dialog)  Indices=[1]  OutputSizes=1  RuntimeRangeChecks=off
  Selector15 : Selector  InputPortWidth=3  IndexOptions=Index vector (dialog)  Indices=2  OutputSizes=1  RuntimeRangeChecks=off
  Selector16 : Selector  InputPortWidth=3  IndexOptions=Index vector (dialog)  Indices=3  OutputSizes=1  RuntimeRangeChecks=off
  Selector18 : Selector  InputPortWidth=3  IndexOptions=Index vector (dialog)  Indices=3  OutputSizes=1  RuntimeRangeChecks=off
  Selector19 : Selector  InputPortWidth=4  IndexOptions=Index vector (dialog)  Indices=[1 2 3]  OutputSizes=1  RuntimeRangeChecks=off
  Selector20 : Selector  InputPortWidth=4  IndexOptions=Index vector (dialog)  Indices=4  OutputSizes=1  RuntimeRangeChecks=off
  Selector22 : Selector  InputPortWidth=4  IndexOptions=Index vector (dialog)  Indices=3  OutputSizes=1  RuntimeRangeChecks=off
  Sub_VelError_Z : Sum  Inputs=+-
  Switch_EnableEKF_IfHovering : Switch  Criteria=u2 > Threshold  SaturateOnIntegerOverflow=off  InputSameDT=off
  Switch_UseNewOrPrevHoverThrust : Switch  Criteria=u2 ~= 0  SaturateOnIntegerOverflow=off  InputSameDT=off
  acc_sp_adjustment : Sum  Inputs=+-
  vel_int_constrain : Subsystem
  hover_thrust_filtered : Outport
  vel_integral_updated_3x1 : Outport  Port=2
  hover_thrust_state : Outport  Port=3
  wires:
  Constant/1 -> Switch_EnableEKF_IfHovering/3, Switch_EnableEKF_IfHovering/1
  dt_s/1 -> HoverThrustEKF_ZeroOrder/3(dt)
  hover_thrust_prev_estimate/1 -> Mul_IntegralUpdate_VelErr_I_dt/2
  accel_sp_z_ms2/1 -> acc_sp_adjustment/2, Sub_VelError_Z/1
  CompareToConst_VelZThreshold/1 -> Switch_EnableEKF_IfHovering/2
  accel_measured_z_ms2/1 -> HoverThrustEKF_ZeroOrder/1(az)
  thrust_body_z_prev/1 -> HoverThrustEKF_ZeroOrder/2(thrust)
  velocity_z_ms/1 -> Selector15/1, Selector14/1, Selector16/1
  gravity_9p81_ms2/1 -> Add_VelIntegral_XY/2, vel_int_constrain/2(integral_upper_limit), Gain4/1, Sub_VelError_Z/2
  Sub_VelError_Z/1 -> Mul_IntegralUpdate_VelErr_I_dt/1
  Switch_UseNewOrPrevHoverThrust/1 -> Assignment6/1, Selector22/1, Selector20/1
  Selector14/1 -> HoverThrustEKF_ZeroOrder/4(vx)
  Selector15/1 -> HoverThrustEKF_ZeroOrder/5(vy)
  Selector16/1 -> HoverThrustEKF_ZeroOrder/6(vz)
  MPC_THR_HOVER_initial/1 -> Mux2/2, HoverThrustEKF_ZeroOrder/7(mpc_hover_thrust)
  Mul_IntegralUpdate_VelErr_I_dt/1 -> Div_ThrustToAccel/1
  Add_VelIntegral_Z/1 -> Assignment5/2
  HoverThrustEKF_ZeroOrder/1(hover_thrust_estimate) -> Div_ThrustToAccel/2, hover_thrust_filtered/1, Mux1/2  "hover_thrust"
  vel_integral_prev_3x1/1 -> Cast To Single/1  "vel_int_in"
  Div_ThrustToAccel/1 -> Add_VelIntegral_XY/1
  Add_VelIntegral_XY/1 -> acc_sp_adjustment/1
  Cast To Single/1 -> Assignment5/1, Selector18/1, Mux2/1
  Gain4/1 -> vel_int_constrain/3(integral_lower_limit)
  vel_int_constrain/1(vel_integral_clamped) -> Assignment6/2
  Selector18/1 -> Add_VelIntegral_Z/1
  acc_sp_adjustment/1 -> Add_VelIntegral_Z/2
  Mux2/1 -> Switch_UseNewOrPrevHoverThrust/3
  Assignment5/1 -> Mux1/1
  Switch_EnableEKF_IfHovering/1 -> Memory/1
  Mux1/1 -> Switch_UseNewOrPrevHoverThrust/1
  Memory/1 -> Switch_UseNewOrPrevHoverThrust/2, CompareToConst_VelZThreshold/1
  Selector20/1 -> hover_thrust_state/1
  Selector22/1 -> vel_int_constrain/1(vel_integral_raw)
  Assignment6/1 -> Selector19/1
  Selector19/1 -> vel_integral_updated_3x1/1  "vel_int"

== system flightControlSystem/MultiCopter Controller/Position & Altitude controller/Position controller/PositionVelocityControl/IgnoreOpticalFlow_till_25cm ==
  note: Keep Velocity X,Y = 0 till drone reaches 25 cm height to avoid reacting to Optical flow noise
  velocity_from_optical_flow : Inport
  altitude_AGL_m : Inport  Port=2
  dt_s : Inport  Port=3
  Assignment : Assignment  DiagnosticForDimensions=Warning  IndexOptions=Index vector (dialog)  Indices=[1,2]  OutputSizes=1  RuntimeRangeChecks=off
  Assignment1 : Assignment  DiagnosticForDimensions=Warning  IndexOptions=Index vector (dialog)  Indices=3  OutputSizes=1
  Constant : Constant  Value=-0.25  SampleTime=-1
  Constant1 : Constant  Value=0  SampleTime=-1
  Relational Operator : RelationalOperator  Operator=>  OutDataTypeStr=boolean  RndMeth=Simplest  InputSameDT=off
  Selector : Selector  InputPortWidth=3  IndexOptions=Index vector (dialog)  Indices=[3]  OutputSizes=1
  Switch : Switch  Criteria=u2 > Threshold  SaturateOnIntegerOverflow=off  InputSameDT=off
  TakeoffRamp_VelZ_Limiter : MATLAB Function  TreatAsAtomicUnit=on
  velocity_flow_gated : Outport
  wires:
  velocity_from_optical_flow/1 -> Switch/3, Assignment/1, Selector/1
  Relational Operator/1 -> Switch/2
  Constant1/1 -> Assignment/2
  Assignment/1 -> Switch/1
  altitude_AGL_m/1 -> Relational Operator/1
  Constant/1 -> Relational Operator/2
  Selector/1 -> TakeoffRamp_VelZ_Limiter/1(vel_sp_z)
  TakeoffRamp_VelZ_Limiter/1(vel_sp_z_limited) -> Assignment1/2
  Assignment1/1 -> velocity_flow_gated/1
  Switch/1 -> Assignment1/1
  dt_s/1 -> TakeoffRamp_VelZ_Limiter/2(dt)

== system flightControlSystem/MultiCopter Controller/Position & Altitude controller/Position controller/PositionVelocityControl/Position P control Loop ==
  note: - Computes position error: pos_error = pos_sp_input - pos
      | - Generates velocity setpoint from position error using
      | proportional gain:
      | vel_sp_position = pos_gain .* pos_error
  vel_sp_feedforward_ms : Inport
  position_setpoint_NED_m : Inport  Port=2
  MPC_XY_VEL_MAX_ms : Inport  Port=3
  MPC_POS_P_gain_3x1 : Inport  Port=4
  position_current_NED_m : Inport  Port=5
  MPC_Z_VEL_MAX_UP_ms : Inport  Port=6
  MPC_Z_VEL_MAX_DN_ms : Inport  Port=7
  Gain : Gain  Gain=-1
  Mux : Mux  Inputs=2
  Product : Product
  Selector : Selector  InputPortWidth=3  IndexOptions=Index vector (dialog)  Indices=[1 2]  OutputSizes=1  RuntimeRangeChecks=off
  Selector1 : Selector  InputPortWidth=3  IndexOptions=Index vector (dialog)  Indices=[1 2]  OutputSizes=1  RuntimeRangeChecks=off
  Selector2 : Selector  InputPortWidth=3  IndexOptions=Index vector (dialog)  Indices=[3]  OutputSizes=1  RuntimeRangeChecks=off
  Subtract : Sum  Inputs=+-
  Subtract1 : Sum  Inputs=+-
  VelSP_Combine_PosError : Subsystem
  constrain : Subsystem
  constrained_xy : Subsystem
  velocity_setpoint_limited_ms : Outport
  wires:
  position_setpoint_NED_m/1 -> Subtract/1
  position_current_NED_m/1 -> Subtract/2
  Subtract/1 -> Product/1  "pos_error"
  MPC_POS_P_gain_3x1/1 -> Product/2
  constrained_xy/1(vel_sp_xy_constrained_ms) -> Mux/1
  MPC_Z_VEL_MAX_UP_ms/1 -> Gain/1
  Selector/1 -> Subtract1/2, constrained_xy/1(vel_sp_xy_2x1)
  constrain/1(vel_sp_z_clamped_ms) -> Mux/2
  Selector1/1 -> Subtract1/1
  Selector2/1 -> constrain/1(vel_sp_z_raw_ms)
  Gain/1 -> constrain/2(neg_MPC_Z_VEL_MAX_UP)
  MPC_Z_VEL_MAX_DN_ms/1 -> constrain/3(MPC_Z_VEL_MAX_DN)
  Subtract1/1 -> constrained_xy/2(vel_sp_feedfwd_xy_2x1)
  MPC_XY_VEL_MAX_ms/1 -> constrained_xy/3(MPC_XY_VEL_MAX_ms)
  Mux/1 -> velocity_setpoint_limited_ms/1
  VelSP_Combine_PosError/2(vel_sp_z_component) -> Selector2/1, Selector1/1
  vel_sp_feedforward_ms/1 -> VelSP_Combine_PosError/1(vel_sp_from_P_gain)
  Product/1 -> VelSP_Combine_PosError/2(vel_sp_feedforward)
  VelSP_Combine_PosError/1(vel_sp_xy_component) -> Selector/1

== system flightControlSystem/MultiCopter Controller/Position & Altitude controller/Position controller/PositionVelocityControl/VelocityError_Computation ==
  MPC_THR_MIN_normalized : Inport
  Constant : Constant  Value=10e-4  SampleTime=-1
  Max : MinMax  Function=max  Inputs=2
  thrust_min_adjusted : Outport
  wires:
  MPC_THR_MIN_normalized/1 -> Max/1
  Constant/1 -> Max/2
  Max/1 -> thrust_min_adjusted/1

== system flightControlSystem/MultiCopter Controller/Position & Altitude controller/Position controller/PositionVelocityControl/Velocity_Control ==
  velocity_error_NED_ms : Inport
  MPC_VEL_P_gain_3x1 : Inport  Port=2
  accel_sp_feedforward_ms2 : Inport  Port=3
  accel_measured_for_Dterm_ms2 : Inport  Port=4
  MPC_VEL_D_gain_3x1 : Inport  Port=5
  vel_integral_state_3x1 : Inport  Port=6
  Mul_Dterm_Accel_x_D : Product
  Mul_Pterm_VelErr_x_P : Product
  Sum_VelPID_AccSP : Sum  Inputs=++-
  addIfNotNan_AccSP_Feedfwd : MATLAB Function  TreatAsAtomicUnit=on
  accel_setpoint_total_ms2 : Outport
  vel_error_for_integral : Outport  Port=2
  wires:
  MPC_VEL_P_gain_3x1/1 -> Mul_Pterm_VelErr_x_P/2
  velocity_error_NED_ms/1 -> vel_error_for_integral/1, Mul_Pterm_VelErr_x_P/1
  accel_measured_for_Dterm_ms2/1 -> Mul_Dterm_Accel_x_D/1
  accel_sp_feedforward_ms2/1 -> addIfNotNan_AccSP_Feedfwd/1("setpoint ")
  MPC_VEL_D_gain_3x1/1 -> Mul_Dterm_Accel_x_D/2
  vel_integral_state_3x1/1 -> Sum_VelPID_AccSP/2
  Mul_Pterm_VelErr_x_P/1 -> Sum_VelPID_AccSP/1
  Mul_Dterm_Accel_x_D/1 -> Sum_VelPID_AccSP/3
  Sum_VelPID_AccSP/1 -> addIfNotNan_AccSP_Feedfwd/2(addition)
  addIfNotNan_AccSP_Feedfwd/1(setpoint) -> accel_setpoint_total_ms2/1

== system flightControlSystem/MultiCopter Controller/Position & Altitude controller/Position controller/PositionVelocityControl/acceleration_control ==
  note: Converts acceleration setpoint to thrust vector, applies tilt and thrust constraints
  accel_setpoint_NED_ms2 : Inport
  hover_thrust_normalized : Inport  Port=2
  MPC_THR_MIN_normalized : Inport  Port=3
  MPC_TILTMAX_AIR_rad : Inport  Port=4
  ACC_Decoupling : Subsystem
  Constant1 : Constant  Value=[0;0;1]  SampleTime=-1
  Constant2 : Constant  Value=9.81  SampleTime=-1
  Constant3 : Constant  Value=[0;0;1]  SampleTime=-1
  Divide : Product  Inputs=*/
  Divide1 : Product  Inputs=*/
  Dot Product : DotProduct  OutDataTypeStr=Inherit: Inherit via internal rule
  Gain1 : Gain  Gain=-1  OutDataTypeStr=double
  Gain2 : Gain  Gain=-1  OutDataTypeStr=double
  Gain_NegateForNED : Gain  Gain=-1
  Min_ThrustFloor : MinMax  Inputs=2
  Mul_AccToThrust_HoverPerG : Product
  Mux_ThrustVector_XYZ : Mux  Inputs=3
  Normalize Vector : vrlib/Utilities/Normalize Vector  maxzero=0
  Product1 : Product
  Selector : Selector  InputPortWidth=3  IndexOptions=Index vector (dialog)  Indices=1  OutputSizes=1  RuntimeRangeChecks=off
  Selector1 : Selector  InputPortWidth=3  IndexOptions=Index vector (dialog)  Indices=2  OutputSizes=1  RuntimeRangeChecks=off
  Selector2 : Selector  InputPortWidth=3  IndexOptions=Index vector (dialog)  Indices=[3]  OutputSizes=1  RuntimeRangeChecks=off
  Sub_AccSP_MinusGravity : Sum  Inputs=+-
  limitTilt : Subsystem
  thrust_setpoint_NED_3x1 : Outport
  accel_sp_after_tilt_limit : Outport  Port=2
  wires:
  MPC_THR_MIN_normalized/1 -> Gain_NegateForNED/1
  Selector/1 -> Gain1/1
  Constant2/1 -> Divide/2
  Gain1/1 -> Mux_ThrustVector_XYZ/1
  accel_setpoint_NED_ms2/1 -> Selector/1, Selector2/1, Selector1/1, accel_sp_after_tilt_limit/1
  Divide/1 -> Mul_AccToThrust_HoverPerG/2
  hover_thrust_normalized/1 -> Sub_AccSP_MinusGravity/2, Divide/1
  Selector2/1 -> ACC_Decoupling/1(thrust_body_previous_3x1), Mul_AccToThrust_HoverPerG/1
  Selector1/1 -> Gain2/1
  Mul_AccToThrust_HoverPerG/1 -> Sub_AccSP_MinusGravity/1
  Gain2/1 -> Mux_ThrustVector_XYZ/2
  Sub_AccSP_MinusGravity/1 -> Divide1/1
  Mux_ThrustVector_XYZ/1 -> Normalize Vector/1
  Normalize Vector/1 -> limitTilt/1(thrust_direction_body)
  Constant1/1 -> limitTilt/2(gravity_direction_NED)
  Min_ThrustFloor/1 -> Product1/2
  MPC_TILTMAX_AIR_rad/1 -> limitTilt/3(MPC_TILTMAX_AIR_rad)
  limitTilt/1(thrust_direction_tilt_limited) -> Product1/1, Dot Product/2
  Constant3/1 -> Dot Product/1
  Dot Product/1 -> Divide1/2
  Divide1/1 -> Min_ThrustFloor/1
  Gain_NegateForNED/1 -> Min_ThrustFloor/2
  Product1/1 -> thrust_setpoint_NED_3x1/1
  ACC_Decoupling/1(tilt_correction_NED_ms2) -> Mux_ThrustVector_XYZ/3

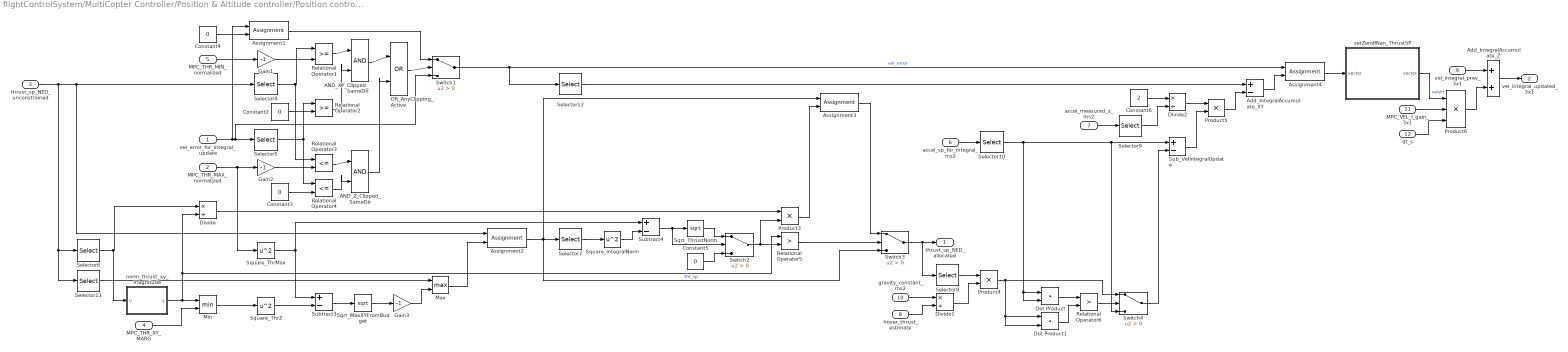
== system flightControlSystem/MultiCopter Controller/Position & Altitude controller/Position controller/PositionVelocityControl/thrust_allocation ==
  vel_error_for_integral_update : Inport
  MPC_THR_MAX_normalized : Inport  Port=2
  thrust_sp_NED_unconstrained : Inport  Port=3
  MPC_THR_XY_MARG : Inport  Port=4
  MPC_THR_MIN_normalized : Inport  Port=5
  accel_sp_for_integral_ms2 : Inport  Port=6
  accel_measured_z_ms2 : Inport  Port=7
  hover_thrust_estimate : Inport  Port=8
  vel_integral_prev_3x1 : Inport  Port=9
  gravity_constant_ms2 : Inport  Port=10
  MPC_VEL_I_gain_3x1 : Inport  Port=11
  dt_s : Inport  Port=12
  AND_XY_Clipped_SameDir : Logic  IconShape=distinctive  AllPortsSameDT=off  OutDataTypeStr=boolean
  AND_Z_Clipped_SameDir : Logic  IconShape=distinctive  AllPortsSameDT=off  OutDataTypeStr=boolean
  Add_IntegralAccumulate_XY : Sum  Inputs=+-
  Add_IntegralAccumulate_Z : Sum
  Assignment1 : Assignment  DiagnosticForDimensions=Warning  IndexOptions=Index vector (dialog)  Indices=3  OutputSizes=1  RuntimeRangeChecks=off
  Assignment2 : Assignment  DiagnosticForDimensions=Warning  IndexOptions=Index vector (dialog)  Indices=3  OutputSizes=1  RuntimeRangeChecks=off
  Assignment3 : Assignment  DiagnosticForDimensions=Warning  IndexOptions=Index vector (dialog)  Indices=[1,2]  OutputSizes=1  RuntimeRangeChecks=off
  Assignment4 : Assignment  DiagnosticForDimensions=Warning  IndexOptions=Index vector (dialog)  Indices=[1 2]  OutputSizes=1  RuntimeRangeChecks=off
  Constant{2..5} (4 alike) : Constant  Value=0  SampleTime=-1
  Constant6 : Constant  Value=2  SampleTime=-1
  Divide : Product  Inputs=*/
  Divide1 : Product  Inputs=*/
  Divide2 : Product  Inputs=*/
  Dot Product : DotProduct  OutDataTypeStr=Inherit: Inherit via internal rule
  Dot Product1 : DotProduct  OutDataTypeStr=Inherit: Inherit via internal rule
  Gain1 : Gain  Gain=-1
  Gain2 : Gain  Gain=-1
  Gain3 : Gain  Gain=-1
  Max : MinMax  Function=max  Inputs=2
  Min : MinMax  Inputs=2
  OR_AnyClipping_Active : Logic  Operator=OR  IconShape=distinctive  AllPortsSameDT=off  OutDataTypeStr=boolean
  Product3 : Product
  Product4 : Product
  Product5 : Product
  Product6 : Product  Inputs=3
  Relational Operator1 : RelationalOperator  OutDataTypeStr=boolean  RndMeth=Simplest  InputSameDT=off
  Relational Operator2 : RelationalOperator  OutDataTypeStr=boolean  RndMeth=Simplest  InputSameDT=off
  Relational Operator3 : RelationalOperator  Operator=<=  OutDataTypeStr=boolean  RndMeth=Simplest  InputSameDT=off
  Relational Operator4 : RelationalOperator  Operator=<=  OutDataTypeStr=boolean  RndMeth=Simplest  InputSameDT=off
  Relational Operator5 : RelationalOperator  Operator=>  OutDataTypeStr=boolean  RndMeth=Simplest  InputSameDT=off
  Relational Operator6 : RelationalOperator  Operator=>  OutDataTypeStr=boolean  RndMeth=Simplest  InputSameDT=off
  Selector{6,8,10,12} (4 alike) : Selector  InputPortWidth=3  IndexOptions=Index vector (dialog)  Indices=[1 2]  OutputSizes=1  RuntimeRangeChecks=off
  Selector{4..5,7,11} (4 alike) : Selector  InputPortWidth=3  IndexOptions=Index vector (dialog)  Indices=3  OutputSizes=1  RuntimeRangeChecks=off
  Selector9 : Selector  InputPortWidth=3  IndexOptions=Index vector (dialog)  Indices=1  OutputSizes=1  RuntimeRangeChecks=off
  Sqrt_MaxXYFromBudget : Sqrt
  Sqrt_ThrustNorm : Sqrt
  Square_IntegralNorm : Math  Operator=square
  Square_ThrMax : Math  Operator=square
  Square_ThrZ : Math  Operator=square
  Sub_VelIntegralUpdate : Sum  Inputs=+-
  Subtract3 : Sum  Inputs=+-
  Subtract4 : Sum  Inputs=+-
  Switch{1..4} (4 alike) : Switch  Criteria=u2 > Threshold  SaturateOnIntegerOverflow=off  InputSameDT=off
  norm_thrust_xy_magnitude : MATLAB Function  TreatAsAtomicUnit=on
  setZeroIfNan_ThrustSP : MATLAB Function  TreatAsAtomicUnit=on
  thrust_sp_NED_allocated : Outport
  vel_integral_updated_3x1 : Outport  Port=2
  wires:
  Assignment2/1 -> Assignment3/1, Switch3/3, Selector7/1  "thr_sp"
  thrust_sp_NED_unconstrained/1 -> Selector6/1, Selector11/1, Selector4/1, Assignment2/1
  Constant4/1 -> Assignment1/2
  norm_thrust_xy_magnitude/1(y) -> Relational Operator5/1, Divide/2, Min/1
  Divide2/1 -> Product5/1
  Min/1 -> Square_ThrZ/1
  Selector6/1 -> Divide/1, norm_thrust_xy_magnitude/1(u)
  Constant6/1 -> Divide2/1
  Selector11/1 -> Max/1
  MPC_THR_XY_MARG/1 -> Min/2
  vel_error_for_integral_update/1 -> Selector5/1, Switch1/3, Assignment1/1
  Selector12/1 -> Add_IntegralAccumulate_XY/1
  MPC_THR_MIN_normalized/1 -> Gain1/1
  MPC_THR_MAX_normalized/1 -> Square_ThrMax/1, Gain2/1
  Switch4/1 -> Sub_VelIntegralUpdate/2
  Divide/1 -> Product3/1
  Assignment1/1 -> Switch1/1
  accel_measured_z_ms2/1 -> Selector9/1
  Gain1/1 -> Relational Operator1/2
  Selector4/1 -> Relational Operator3/1, Relational Operator1/1
  Constant2/1 -> Relational Operator2/2
  Selector5/1 -> Relational Operator4/1, Relational Operator2/1
  Gain2/1 -> Relational Operator3/2
  Relational Operator6/1 -> Switch4/2
  Switch2/1 -> Product3/2, Relational Operator5/2
  Constant3/1 -> Relational Operator4/2
  Square_ThrMax/1 -> Subtract4/1, Subtract3/1
  Square_ThrZ/1 -> Subtract3/2
  Relational Operator1/1 -> AND_XY_Clipped_SameDir/1
  Relational Operator2/1 -> AND_XY_Clipped_SameDir/2
  Relational Operator3/1 -> AND_Z_Clipped_SameDir/1
  Relational Operator4/1 -> AND_Z_Clipped_SameDir/2
  Subtract3/1 -> Sqrt_MaxXYFromBudget/1
  AND_XY_Clipped_SameDir/1 -> OR_AnyClipping_Active/1
  AND_Z_Clipped_SameDir/1 -> OR_AnyClipping_Active/2
  Sqrt_MaxXYFromBudget/1 -> Gain3/1
  Add_IntegralAccumulate_Z/1 -> vel_integral_updated_3x1/1
  OR_AnyClipping_Active/1 -> Switch1/2
  Product5/1 -> Add_IntegralAccumulate_XY/2
  Gain3/1 -> Max/2
  Switch1/1 -> Assignment4/1, Selector12/1  "vel_error"
  Divide1/1 -> Product4/2
  Max/1 -> Assignment2/2
  Selector7/1 -> Square_IntegralNorm/1
  Square_IntegralNorm/1 -> Subtract4/2
  Subtract4/1 -> Switch2/2, Sqrt_ThrustNorm/1
  Sqrt_ThrustNorm/1 -> Switch2/1
  Constant5/1 -> Switch2/3
  Selector9/1 -> Divide2/2
  Product3/1 -> Assignment3/2
  accel_sp_for_integral_ms2/1 -> Selector10/1
  Relational Operator5/1 -> Switch3/2
  Assignment3/1 -> Switch3/1
  Switch3/1 -> thrust_sp_NED_allocated/1, Selector8/1
  Selector10/1 -> Dot Product/2, Dot Product/1, Switch4/3, Sub_VelIntegralUpdate/1
  gravity_constant_ms2/1 -> Divide1/1
  hover_thrust_estimate/1 -> Divide1/2
  Product4/1 -> Dot Product1/2, Dot Product1/1, Switch4/1
  Selector8/1 -> Product4/1
  Dot Product/1 -> Relational Operator6/1
  Dot Product1/1 -> Relational Operator6/2
  Sub_VelIntegralUpdate/1 -> Product5/2
  Add_IntegralAccumulate_XY/1 -> Assignment4/2
  Assignment4/1 -> setZeroIfNan_ThrustSP/1("vector ")
  setZeroIfNan_ThrustSP/1(vector) -> Product6/1  "velerr"
  MPC_VEL_I_gain_3x1/1 -> Product6/2
  dt_s/1 -> Product6/3
  vel_integral_prev_3x1/1 -> Add_IntegralAccumulate_Z/1
  Product6/1 -> Add_IntegralAccumulate_Z/2

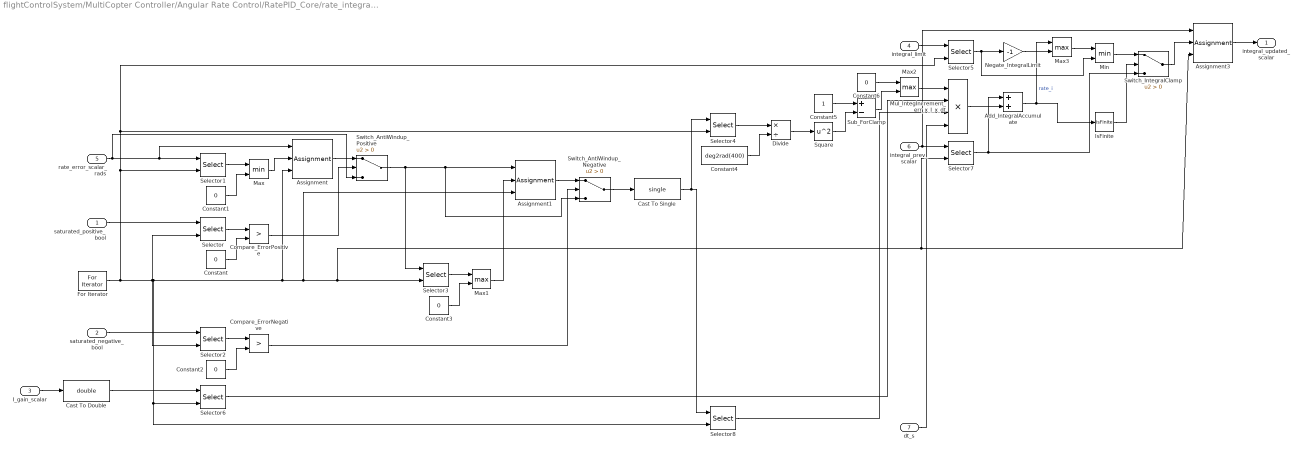
== system flightControlSystem/MultiCopter Controller/Angular Rate Control/RatePID_Core/rate_integral/AntiWindup_IntegralUpdate/Update_Integral ==
  saturated_positive_bool : Inport
  saturated_negative_bool : Inport  Port=2
  I_gain_scalar : Inport  Port=3
  integral_limit : Inport  Port=4
  rate_error_scalar_rads : Inport  Port=5
  integral_prev_scalar : Inport  Port=6
  dt_s : Inport  Port=7
  Add_IntegralAccumulate : Sum
  Assignment : Assignment  DiagnosticForDimensions=Warning  IndexOptions=Index vector (port)  Indices=1  OutputSizes=1  RuntimeRangeChecks=off
  Assignment1 : Assignment  DiagnosticForDimensions=Warning  IndexOptions=Index vector (port)  Indices=1  OutputSizes=1  RuntimeRangeChecks=off
  Assignment3 : Assignment  DiagnosticForDimensions=Warning  IndexOptions=Index vector (port)  Indices=1  OutputSizes=1  RuntimeRangeChecks=off
  Cast To Double : DataTypeConversion  OutDataTypeStr=double  SaturateOnIntegerOverflow=off  RndMeth=Floor
  Cast To Single : DataTypeConversion  OutDataTypeStr=single  SaturateOnIntegerOverflow=off  RndMeth=Floor
  Compare_ErrorNegative : RelationalOperator  Operator=>  OutDataTypeStr=boolean  RndMeth=Simplest  InputSameDT=off
  Compare_ErrorPositive : RelationalOperator  Operator=>  OutDataTypeStr=boolean  RndMeth=Simplest  InputSameDT=off
  Constant{,1..3,6} (5 alike) : Constant  Value=0  SampleTime=-1
  Constant4 : Constant  Value=deg2rad(400)  SampleTime=-1
  Constant5 : Constant  SampleTime=-1
  Divide : Product  Inputs=*/
  For Iterator : ForIterator  IterationLimit=3
  IsFinite : RelationalOperator  Operator=isFinite  OutDataTypeStr=boolean  RndMeth=Simplest  InputSameDT=off
  Max : MinMax  Inputs=2
  Max1 : MinMax  Function=max  Inputs=2  OutDataTypeStr=double
  Max2 : MinMax  Function=max  Inputs=2
  Max3 : MinMax  Function=max  Inputs=2
  Min : MinMax  Inputs=2
  Mul_IntegIncrement_err_x_I_x_dt : Product  Inputs=4
  Negate_IntegralLimit : Gain  Gain=-1
  Selector{,1..8} (9 alike) : Selector  InputPortWidth=3  IndexOptions=Index vector (port)  Indices=[1 3]  OutputSizes=1  RuntimeRangeChecks=off
  Square : Math  Operator=square
  Sub_ForClamp : Sum  Inputs=+-
  Switch_AntiWindup_Negative : Switch  Criteria=u2 > Threshold  SaturateOnIntegerOverflow=off  InputSameDT=off
  Switch_AntiWindup_Positive : Switch  Criteria=u2 > Threshold  SaturateOnIntegerOverflow=off  InputSameDT=off
  Switch_IntegralClamp : Switch  Criteria=u2 > Threshold  SaturateOnIntegerOverflow=off  InputSameDT=off
  integral_updated_scalar : Outport
  wires:
  Switch_AntiWindup_Positive/1 -> Switch_AntiWindup_Negative/3, Assignment1/1, Selector3/1
  I_gain_scalar/1 -> Cast To Double/1
  rate_error_scalar_rads/1 -> Assignment/1, Selector1/1, Switch_AntiWindup_Positive/3
  Selector1/1 -> Max/1
  Selector7/1 -> Switch_IntegralClamp/3, Add_IntegralAccumulate/1
  saturated_positive_bool/1 -> Selector/1
  Constant1/1 -> Max/2
  Sub_ForClamp/1 -> Max2/2
  saturated_negative_bool/1 -> Selector2/1
  For Iterator/1 -> Selector8/2, Selector6/2, Selector7/2, Assignment3/3, Selector3/2, Assignment1/3, Assignment/3, Selector2/2, Selector/2, Selector4/2, Selector5/2, Selector1/2
  Selector/1 -> Compare_ErrorPositive/1
  Cast To Double/1 -> Selector6/1
  Constant/1 -> Compare_ErrorPositive/2
  Selector2/1 -> Compare_ErrorNegative/1
  Constant2/1 -> Compare_ErrorNegative/2
  Selector6/1 -> Mul_IntegIncrement_err_x_I_x_dt/2
  Max/1 -> Assignment/2
  Compare_ErrorPositive/1 -> Switch_AntiWindup_Positive/2
  Compare_ErrorNegative/1 -> Switch_AntiWindup_Negative/2
  Assignment3/1 -> integral_updated_scalar/1
  Assignment/1 -> Switch_AntiWindup_Positive/1
  Selector3/1 -> Max1/1
  Constant3/1 -> Max1/2
  Max1/1 -> Assignment1/2
  Assignment1/1 -> Switch_AntiWindup_Negative/1
  Switch_AntiWindup_Negative/1 -> Cast To Single/1
  Cast To Single/1 -> Selector8/1, Selector4/1
  integral_limit/1 -> Selector5/1
  Selector4/1 -> Divide/1
  Constant4/1 -> Divide/2
  IsFinite/1 -> Switch_IntegralClamp/2
  Selector8/1 -> Mul_IntegIncrement_err_x_I_x_dt/3
  Divide/1 -> Square/1
  Constant5/1 -> Sub_ForClamp/1
  Square/1 -> Sub_ForClamp/2
  Constant6/1 -> Max2/1
  Max2/1 -> Mul_IntegIncrement_err_x_I_x_dt/1
  integral_prev_scalar/1 -> Assignment3/1, Selector7/1
  dt_s/1 -> Mul_IntegIncrement_err_x_I_x_dt/4
  Selector5/1 -> Min/2, Negate_IntegralLimit/1
  Mul_IntegIncrement_err_x_I_x_dt/1 -> Add_IntegralAccumulate/2
  Negate_IntegralLimit/1 -> Max3/2
  Add_IntegralAccumulate/1 -> Max3/1, IsFinite/1  "rate_i"
  Max3/1 -> Min/1
  Min/1 -> Switch_IntegralClamp/1
  Switch_IntegralClamp/1 -> Assignment3/2

== system flightControlSystem/MultiCopter Controller/Position & Altitude controller/Position controller/PositionVelocityControl/Hover_Thrust/vel_int_constrain ==
  vel_integral_raw : Inport
  integral_upper_limit : Inport  Port=2
  integral_lower_limit : Inport  Port=3
  Max : MinMax  Function=max  Inputs=2
  Min : MinMax  Inputs=2
  vel_integral_clamped : Outport
  wires:
  vel_integral_raw/1 -> Max/1
  integral_lower_limit/1 -> Max/2
  Max/1 -> Min/1
  integral_upper_limit/1 -> Min/2
  Min/1 -> vel_integral_clamped/1

== system flightControlSystem/MultiCopter Controller/Position & Altitude controller/Position controller/PositionVelocityControl/Position P control Loop/VelSP_Combine_PosError ==
  vel_sp_from_P_gain : Inport
  vel_sp_feedforward : Inport  Port=2
  addIfNotNan_VelSP_Plus_Feedfwd : MATLAB Function  TreatAsAtomicUnit=on
  setZeroIfNan_VelSP : MATLAB Function  TreatAsAtomicUnit=on
  vel_sp_xy_component : Outport
  vel_sp_z_component : Outport  Port=2
  wires:
  vel_sp_feedforward/1 -> setZeroIfNan_VelSP/1("vector "), addIfNotNan_VelSP_Plus_Feedfwd/2(addition)
  addIfNotNan_VelSP_Plus_Feedfwd/1(setpoint) -> vel_sp_z_component/1
  vel_sp_from_P_gain/1 -> addIfNotNan_VelSP_Plus_Feedfwd/1("setpoint ")
  setZeroIfNan_VelSP/1(vector) -> vel_sp_xy_component/1
